simulink model "Five_Level_Inverter"  (R2025a)
settings: Solver=FixedStepAuto  StartTime=0.0  StopTime=0.5  RelTol=1e-3
undefined symbols (not defined in the file): fc, Ts
libraries: spsIGBTDiodeLib x8, simulink x4, spsDCVoltageSourceLib x2, spsCurrentMeasurementLib x1, spsSeriesRLCBranchLib x1, sps_lib x1
settings Model: Creator=HP  LastModifiedBy=HP
settings DataIOCC: SaveFormat=StructureWithTime  ReturnWorkspaceOutputs=off
settings RTWCC: RTWVerbose=off

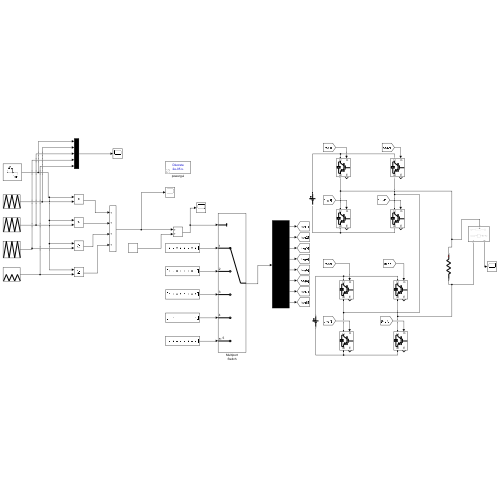
[thumbnail: Simulink's stored preview of the top-level diagram]
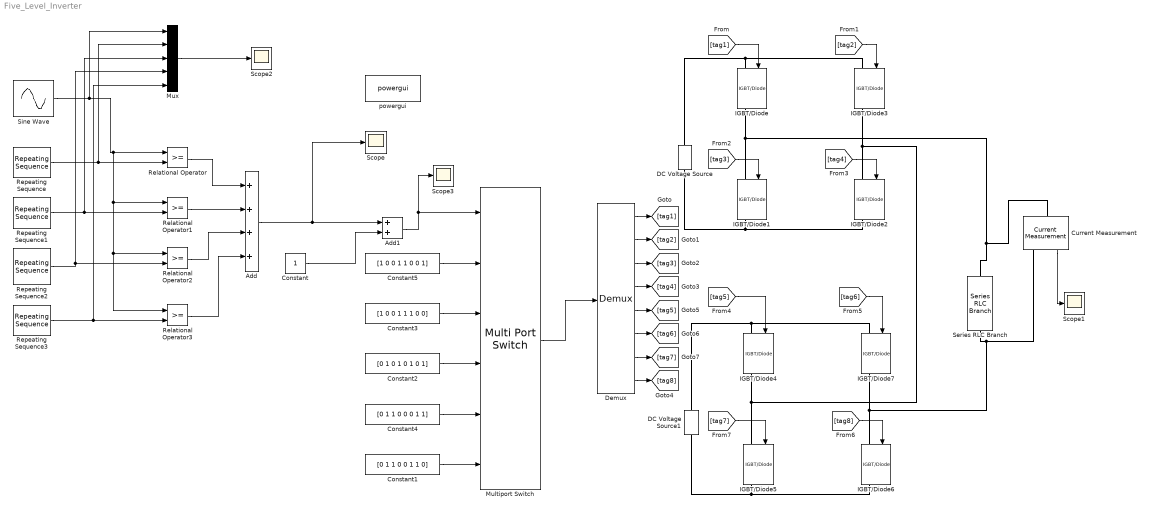
== system Five_Level_Inverter ==
  Add : Sum  Inputs=++++
  Add1 : Sum
  Constant : Constant
  Constant1 : Constant  Value=[0 1 1 0 0 1 1 0]
  Constant2 : Constant  Value=[0 1 0 1 0 1 0 1]
  Constant3 : Constant  Value=[1 0 0 1 1 1 0 0]
  Constant4 : Constant  Value=[0 1 1 0 0 0 1 1]
  Constant5 : Constant  Value=[1 0 0 1 1 0 0 1]
  Current Measurement : spsCurrentMeasurementLib/Current Measurement  PhasorSimulation=off  OutputType=Complex  PSBequivalent=0
  DC Voltage Source : spsDCVoltageSourceLib/DC Voltage Source  Amplitude=100  Measurements=None
  DC Voltage Source1 : spsDCVoltageSourceLib/DC Voltage Source  Amplitude=100  Measurements=None
  Demux : Demux  Outputs=8
  IGBT/Diode{,1..7} (8 alike) : spsIGBTDiodeLib/IGBT//Diode  Ron=1e-3  Rs=1e5  Cs=inf  Measurements=on
  Multiport Switch : MultiPortSwitch  Inputs=5  SaturateOnIntegerOverflow=off  InputSameDT=off
  Mux : Mux  Inputs=5
  Relational Operator{,1..3} (4 alike) : RelationalOperator  OutDataTypeStr=boolean  RndMeth=Simplest  InputSameDT=off
  Repeating Sequence : simulink/Sources/Repeating Sequence  rep_seq_t=[0 0.5/fc 1/fc]  rep_seq_y=[1 2 1]
  Repeating Sequence1 : simulink/Sources/Repeating Sequence  rep_seq_t=[0 0.5/fc 1/fc]  rep_seq_y=[0 1 0]
  Repeating Sequence2 : simulink/Sources/Repeating Sequence  rep_seq_t=[0 0.5/fc 1/fc]  rep_seq_y=[-1 0 -1]
  Repeating Sequence3 : simulink/Sources/Repeating Sequence  rep_seq_t=[0 0.5/fc 1/fc]  rep_seq_y=[-2 -1 -2]
  Scope{,1..3} (4 alike) : Scope
      Scope settings: ActiveDisplayYMinimum=-0.61962324383973488  ActiveDisplayYMaximum=4.6029566345856585
      Scope1 settings: ActiveDisplayYMinimum=-62499.99990080639  ActiveDisplayYMaximum=62499.999431398042  DataLoggingVariableName=Vo
      Scope2 settings: ActiveDisplayYMinimum=-2.2789434658309684  ActiveDisplayYMaximum=2.2582744982687877  DataLoggingVariableName=ScopeData2
      Scope3 settings: ActiveDisplayYMinimum=0.50000000000000011  ActiveDisplayYMaximum=5.5  DataLoggingVariableName=ScopeData3
  Series RLC Branch : spsSeriesRLCBranchLib/Series RLC Branch  LConnTagsString=__new0  RConnTagsString=__new0  BranchType=R  Resistance=100  Inductance=1e-3  SetiL0=off  InitialCurrent=0  Capacitance=1e-6  Setx0=off  InitialVoltage=0  Measurements=None
  Sine Wave : Sin  Amplitude=1.9  Frequency=2*pi*50  SampleTime=Ts
  powergui : sps_lib/powergui  Priority=1  SimulationMode=Discrete  SampleTime=20e-6  frequency=60  Iterations=50  frequencyindice=0  Pbase=100e6  ErrMax=1e-4  UnitsV=kV  UnitsW=MW  buscounter=0  FunctionMessages=off  echomessages=off  EnableUseOfTLC=off  CurrentSourceSwitches=off  DisableSnubberDevices=off  DisableRonSwitches=off  DisableVfSwitches=off  DisplayEquations=off  AutomaticDiscreteSolvers=off  SolverType=Tustin/Backward Euler (TBE)  Interpol=off  ExternalGateDelay=off  methode=off  Ts=100  x0status=blocks  SPID=on  SwTol=0  HookPort=off  NonlinearTolerance=1e-4  nMaxIteration=100  ContinueOnMaxIteration=off  RestoreLinks=warning  ResistiveCurrentMeasurement=off  Frange=[0:2:500]  Ylog=off  Xlog=on  ShowGrid=off  save=off  variable=ZData  structure=0  ZoomFFT=off  StartTime=0.0  cycles=1  DisplayStyle=1  fundamental=60  FreqAxis=off  MaxFrequency=1000  frequencyindicesteady=1  RmsSteady=1  display=off
  wires:
  Repeating Sequence/1 -> Mux/2, Relational Operator/2
  Repeating Sequence1/1 -> Mux/3, Relational Operator1/2
  Repeating Sequence2/1 -> Mux/4, Relational Operator2/2
  Repeating Sequence3/1 -> Mux/5, Relational Operator3/2
  Sine Wave/1 -> Mux/1, Relational Operator3/1, Relational Operator2/1, Relational Operator1/1, Relational Operator/1
  Relational Operator/1 -> Add/1
  Relational Operator1/1 -> Add/2
  Relational Operator2/1 -> Add/3
  Relational Operator3/1 -> Add/4
  Add/1 -> Scope/1, Add1/1
  Constant/1 -> Add1/2
  Multiport Switch/1 -> Demux/1
  Add1/1 -> Scope3/1, Multiport Switch/1
  Constant1/1 -> Multiport Switch/6
  Demux/1 -> [tag1]
  Constant2/1 -> Multiport Switch/4
  Constant4/1 -> Multiport Switch/5
  Constant5/1 -> Multiport Switch/2
  Mux/1 -> Scope2/1
  [tag1] -> IGBT/Diode/1
  Demux/2 -> [tag2]
  [tag2] -> IGBT/Diode3/1
  Demux/3 -> [tag3]
  Demux/8 -> [tag8]
  Demux/4 -> [tag4]
  Demux/5 -> [tag5]
  Demux/6 -> [tag6]
  Demux/7 -> [tag7]
  [tag3] -> IGBT/Diode1/1
  [tag4] -> IGBT/Diode2/1
  [tag5] -> IGBT/Diode4/1
  [tag6] -> IGBT/Diode7/1
  [tag7] -> IGBT/Diode5/1
  [tag8] -> IGBT/Diode6/1
  Constant3/1 -> Multiport Switch/3
  Current Measurement/1 -> Scope1/1
  connections:
  DC Voltage Source/RConn1 -- IGBT/Diode3/LConn1 -- IGBT/Diode/LConn1
  DC Voltage Source/LConn1 -- IGBT/Diode2/RConn1 -- IGBT/Diode1/RConn1
  DC Voltage Source1/RConn1 -- IGBT/Diode7/LConn1 -- IGBT/Diode4/LConn1
  DC Voltage Source1/LConn1 -- IGBT/Diode6/RConn1 -- IGBT/Diode5/RConn1
  IGBT/Diode7/RConn1 -- Current Measurement/RConn1 -- Series RLC Branch/RConn1 -- IGBT/Diode6/LConn1
  IGBT/Diode3/RConn1 -- IGBT/Diode5/LConn1 -- IGBT/Diode4/RConn1 -- IGBT/Diode2/LConn1
  IGBT/Diode/RConn1 -- Current Measurement/LConn1 -- Series RLC Branch/LConn1 -- IGBT/Diode1/LConn1
